simulink model "W07_openloop"  (R2024b)
settings: Solver=ode4  StartTime=0  StopTime=T_final  FixedStep=h  RelTol=1e-3
InitFcn:
  | addpath(fullfile(fileparts(fileparts(fileparts(get_param(bdroot, 'FileName')))), '_tools'), fileparts(get_param(bdroot, 'FileName'))); run_alone('W07', bdroot);
StopFcn:
  | W07_plot;
values from neighbouring files (symbols this model uses):
  alpha_lim = cfg.alpha_max(1)    [W07_0_setup.m]
  alpha_rate = cfg.alpha_rlim(1)    [W07_0_setup.m]
  animate = 1    [W07_0_setup.m]    (also in W07_alloc_run.m = 0; W07_pose_run.m = 0; W07_wpt_run.m = 0)
  beta_c = pi/2    (= 1.57079632679)    [W07_0_setup.m]
  d_cmd = deg2rad(d_deg)    [W07_0_setup.m]    (also in W07_openloop_run.m)
  h = 0.02    [W07_0_setup.m]    (also in W07_3_build_wpt.m = add_line(sys, [a; via; b]); W07_4_build_pose.m = add_line(sys, [a; via; b]))
  mp = 25    [W07_0_setup.m]
  n_cmd = [60 60 60 60]'    [W07_0_setup.m]    (also in W07_openloop_run.m = S{1,2}')
  n_max = cfg.n_max    [W07_0_setup.m]    (also in W07_plot_ca.m = base_num('n_max',      103.93); W07_plot_sat.m = base_var('n_max',      103.931))
  n_min = cfg.n_min    [W07_0_setup.m]    (also in W07_plot_ca.m = base_num('n_min',     -101.74); W07_plot_sat.m = base_var('n_min',     -101.737))
  quad = [cfg.pos ; cfg.alpha_max ; cfg.mount]    [W07_0_setup.m]
  rp = [0.05 0 -0.35]'    [W07_0_setup.m]
  V_c = 0.0    (= 0)    [W07_0_setup.m]
  x0 = zeros(12,1)    [W07_0_setup.m]
settings Model: Creator=admin  LastModifiedBy=wkyou
settings DataIOCC: ReturnWorkspaceOutputs=off

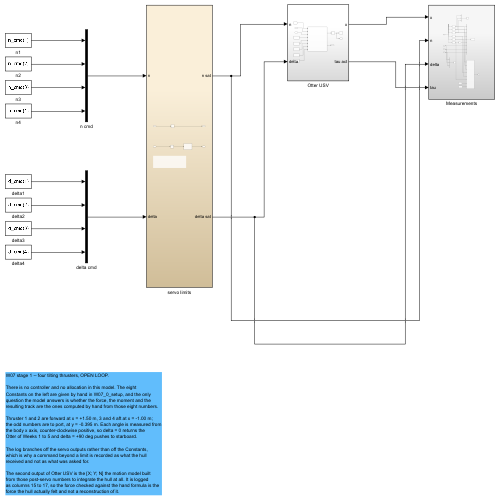
[thumbnail: Simulink's stored preview of the top-level diagram]
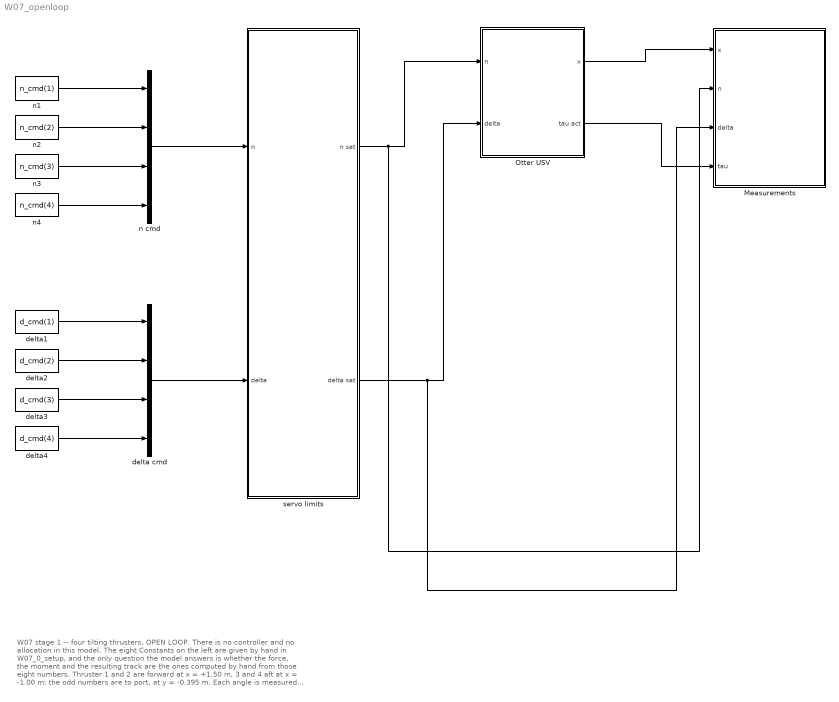
== system W07_openloop ==
  note: W07 stage 1 -- four tilting thrusters, OPEN LOOP.
      |
      | There is no controller and no allocation in this model. The eight
      | Constants on the left are given by hand in W07_0_setup, and the only
      | question the model answers is whether the force, the moment and the
      | resulting track are the ones computed by hand from those eight numbers.
      |
      | Thruster 1 and 2 are forward at x = +1.50 m, 3 and 4 aft at x = -1.00 m;
      | the odd numbers are to port, at y = -0.395 m. Each angle is measured from
      | the body x axis, counter-clockwise positive, so delta = 0 returns the
      | Otter of Weeks 1 to 5 and delta = +90 deg pushes to starboard.
      |
      | The log branches off the servo outputs rather than off the Constants,
      | which is why a command beyond a limit is recorded as what the hull
      | received and not as what was asked for.
      |
      | The second output of Otter USV is the [X; Y; N] the motion model built
      | from those post-servo numbers to integrate the hull at all. It is logged
      | as columns 15 to 17, so the force checked against the hand formula is the
      | force the hull actually felt and not a reconstruction of it.
  Measurements : Subsystem
  Otter USV : Subsystem
  delta cmd : Mux
  delta1 : Constant  Value=d_cmd(1)
  delta2 : Constant  Value=d_cmd(2)
  delta3 : Constant  Value=d_cmd(3)
  delta4 : Constant  Value=d_cmd(4)
  n cmd : Mux
  n1 : Constant  Value=n_cmd(1)
  n2 : Constant  Value=n_cmd(2)
  n3 : Constant  Value=n_cmd(3)
  n4 : Constant  Value=n_cmd(4)
  servo limits : Subsystem
  wires:
  n cmd/1 -> servo limits/1(n)
  delta cmd/1 -> servo limits/2(delta)
  n1/1 -> n cmd/1
  n2/1 -> n cmd/2
  n3/1 -> n cmd/3
  n4/1 -> n cmd/4
  delta1/1 -> delta cmd/1
  delta2/1 -> delta cmd/2
  delta3/1 -> delta cmd/3
  delta4/1 -> delta cmd/4
  servo limits/1(n sat) -> Otter USV/1(n), Measurements/2(n)
  servo limits/2(delta sat) -> Otter USV/2(delta), Measurements/3(delta)
  Otter USV/1(x) -> Measurements/1(x)
  Otter USV/2(tau act) -> Measurements/4(tau)

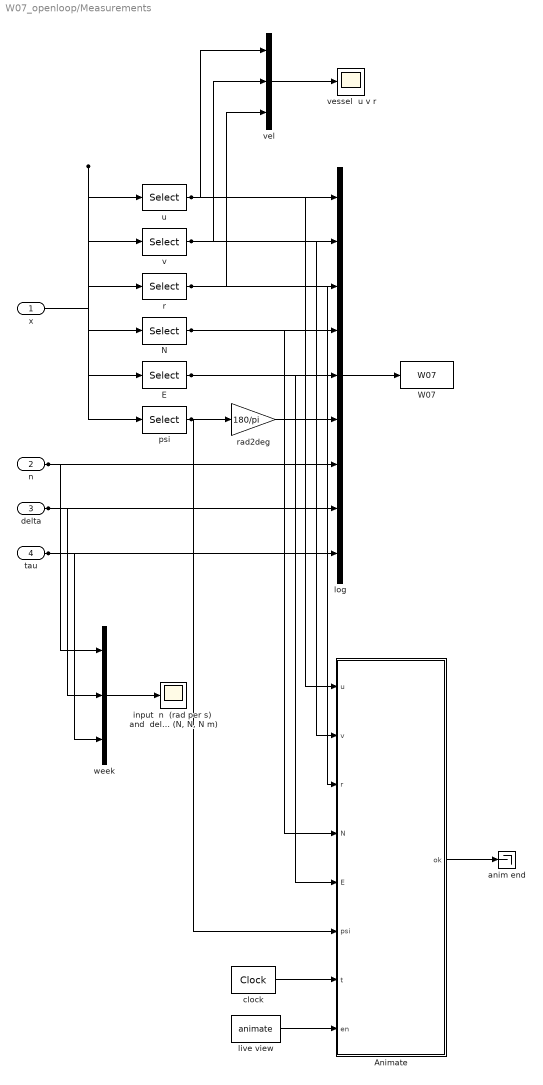
== system W07_openloop/Measurements ==
  x : Inport
  n : Inport  Port=2
  delta : Inport  Port=3
  tau : Inport  Port=4
  Animate : MATLAB Function  TreatAsAtomicUnit=on
  E : Selector  InputPortWidth=12  IndexOptions=Index vector (dialog)  Indices=8  OutputSizes=1
  N : Selector  InputPortWidth=12  IndexOptions=Index vector (dialog)  Indices=7  OutputSizes=1
  W07 : ToWorkspace  VariableName=W07  SaveFormat=Structure With Time  SampleTime=-1
  anim end : Terminator
  clock : DigitalClock  SampleTime=h
  "input  n  (rad per s)  and  delta  (rad),  force delivered  tau  (N, N, N m)" : Scope
  live view : Constant  Value=animate
  log : Mux  Inputs=9
  psi : Selector  InputPortWidth=12  IndexOptions=Index vector (dialog)  Indices=12  OutputSizes=1
  r : Selector  InputPortWidth=12  IndexOptions=Index vector (dialog)  Indices=6  OutputSizes=1
  rad2deg : Gain  Gain=180/pi
  u : Selector  InputPortWidth=12  IndexOptions=Index vector (dialog)  Indices=1  OutputSizes=1
  v : Selector  InputPortWidth=12  IndexOptions=Index vector (dialog)  Indices=2  OutputSizes=1
  vel : Mux  Inputs=3
  vessel  u v r : Scope
  week : Mux  Inputs=3
  wires:
  x/1 -> u/1, v/1, r/1, N/1, E/1, psi/1
  log/1 -> W07/1
  psi/1 -> rad2deg/1, Animate/6(psi)
  u/1 -> log/1, vel/1, Animate/1(u)
  v/1 -> log/2, vel/2, Animate/2(v)
  r/1 -> log/3, vel/3, Animate/3(r)
  N/1 -> log/4, Animate/4(N)
  E/1 -> log/5, Animate/5(E)
  rad2deg/1 -> log/6
  n/1 -> log/7, week/1
  delta/1 -> log/8, week/2
  tau/1 -> log/9, week/3
  vel/1 -> vessel  u v r/1
  week/1 -> "input  n  (rad per s)  and  delta  (rad),  force delivered  tau  (N, N, N m)"/1
  clock/1 -> Animate/7(t)
  live view/1 -> Animate/8(en)
  Animate/1(ok) -> anim end/1

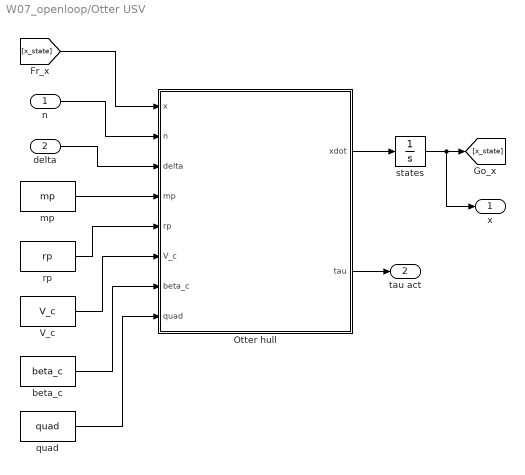
== system W07_openloop/Otter USV ==
  n : Inport
  delta : Inport  Port=2
  Otter hull : MATLAB Function  TreatAsAtomicUnit=on
  V_c : Constant  Value=V_c
  beta_c : Constant  Value=beta_c
  mp : Constant  Value=mp
  quad : Constant  Value=quad
  rp : Constant  Value=rp
  states : Integrator  InitialCondition=x0
  x : Outport
  tau act : Outport  Port=2
  wires:
  [x_state] -> Otter hull/1(x)
  quad/1 -> Otter hull/8(quad)
  delta/1 -> Otter hull/3(delta)
  beta_c/1 -> Otter hull/7(beta_c)
  n/1 -> Otter hull/2(n)
  mp/1 -> Otter hull/4(mp)
  rp/1 -> Otter hull/5(rp)
  V_c/1 -> Otter hull/6(V_c)
  Otter hull/1(xdot) -> states/1
  Otter hull/2(tau) -> tau act/1
  states/1 -> [x_state], x/1

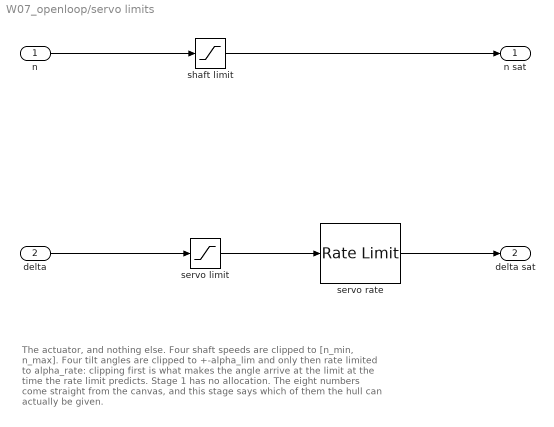
== system W07_openloop/servo limits ==
  note: The actuator, and nothing else.
      |
      | Four shaft speeds are clipped to [n_min, n_max]. Four tilt angles are
      | clipped to +-alpha_lim and only then rate limited to alpha_rate: clipping
      | first is what makes the angle arrive at the limit at the time the rate
      | limit predicts.
      |
      | Stage 1 has no allocation. The eight numbers come straight from the
      | canvas, and this stage says which of them the hull can actually be given.
  n : Inport
  delta : Inport  Port=2
  servo limit : Saturate  UpperLimit=alpha_lim  LowerLimit=-alpha_lim
  servo rate : RateLimiter  RisingSlewLimit=alpha_rate  FallingSlewLimit=-alpha_rate  SampleTimeMode=inherited
  shaft limit : Saturate  UpperLimit=n_max  LowerLimit=n_min
  n sat : Outport
  delta sat : Outport  Port=2
  wires:
  n/1 -> shaft limit/1
  shaft limit/1 -> n sat/1
  delta/1 -> servo limit/1
  servo limit/1 -> servo rate/1
  servo rate/1 -> delta sat/1

== matlab function W07_openloop/Measurements/Animate ==
  data: u input; ok output; v input; r input; N input; E input; psi input; t input; en input
function ok = Animate(u, v, r, N, E, psi, t, en)
%#codegen
% Live view of the vessel while the model runs.
%
% A MATLAB Function block cannot plot, so the drawing function is declared
% extrinsic: Simulink calls plain MATLAB rather than generating code for it.
% Set animate = 0 in the setup script to switch the live view off.
%
% psi arrives in RADIANS and r in rad/s - the units otter.m works in. The
% wrapper converts them for display, in one place, so no two figures in the
% course can disagree about what a degree is.
coder.extrinsic('W07_animate');
ok = 1;
if en > 0.5
    W07_animate(u, v, r, N, E, psi, t);
end
end

== matlab function W07_openloop/Otter USV/Otter hull ==
  data: x input; xdot output double size=[12 1]; n input; delta input; mp input; rp input; V_c input; beta_c input; quad input; tau output double size=[3 1]
function [xdot, tau] = otter_hull(x, n, delta, mp, rp, V_c, beta_c, quad)
% otter_tilt4.m: Fossen's otter.m with four tilting thrusters, called
% unchanged from _tools. Four shaft speeds and four angles in, tau built
% inside, in the same four marked places as otter_bow.m.
%
%   x      12 states, fed back from the integrator
%   n      shaft speeds [rad/s], fore port / fore stbd / aft port / aft stbd
%   delta  tilt angles [rad], measured from the body x axis, CCW positive
%   quad   3 x 4: the x stations, the y stations and the tilt limits
%
% Rows 1, 2 and 6 of tau all carry the angles, by the column rule
% [e_x; e_y; x e_y - y e_x] with e = [cos delta; sin delta]. Nothing is
% added after the call; there is no superposition and no tau_ext port.
%
% The second output is the [X; Y; N] the model actually used, formed after n
% and delta are clipped to their limits. It is the delivered force, so no
% block outside has to rebuild it from n and delta.
%
% otter_tilt4.m is not written for code generation, so the call is extrinsic
% and both outputs have to be pre-sized for Simulink to know their widths.
coder.extrinsic('otter_tilt4');

xdot = zeros(12,1);
spd  = 0;
tau  = zeros(3,1);
[xdot, spd, tau] = otter_tilt4(x, n, delta, mp, rp, V_c, beta_c, quad);
end
